simulink model "TorqueSteerCompensator"  (R2025b)
settings: Solver=VariableStepAuto  StartTime=0.0  StopTime=10.0  RelTol=1e-3
values from neighbouring files (symbols this model uses):
  Ke = 0.8    [TorqueSteerCompensator.mat]
  Kfb = 0.5    [TorqueSteerCompensator.mat]
  Kff = 1    [TorqueSteerCompensator.mat]
settings Model: Creator=sharm  LastModifiedBy=sharm

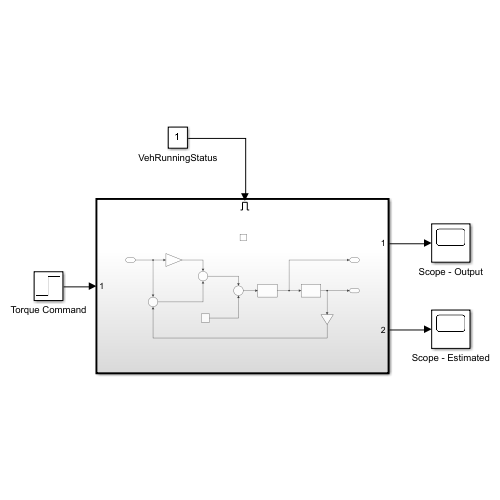
[thumbnail: Simulink's stored preview of the top-level diagram]
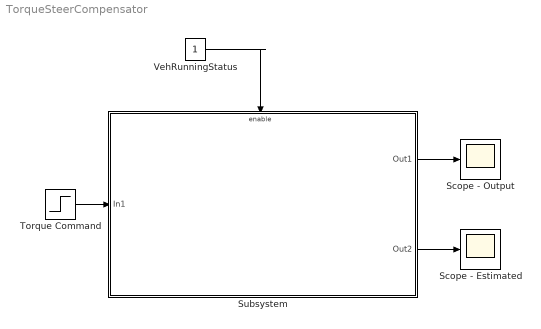
== system TorqueSteerCompensator ==
  Scope - Estimated : Scope
      settings: ActiveDisplayYMinimum=-0.16435887299849231  ActiveDisplayYMaximum=1.4792298569864311
  Scope - Output : Scope
      settings: ActiveDisplayYMinimum=-0.3828039560539751  ActiveDisplayYMaximum=1.9112315071928312
  Subsystem : Subsystem
  Torque Command : Step  SampleTime=0
  VehRunningStatus : Constant
  wires:
  Torque Command/1 -> Subsystem/1(In1)
  Subsystem/1(Out1) -> Scope - Output/1
  Subsystem/2(Out2) -> Scope - Estimated/1
  VehRunningStatus/1 -> Subsystem/Enable

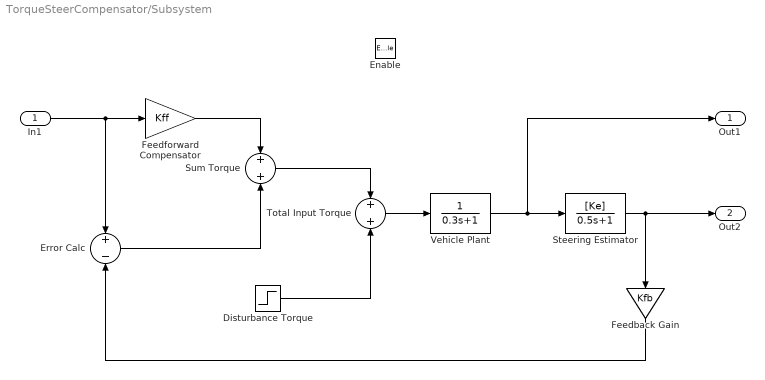
== system TorqueSteerCompensator/Subsystem ==
  In1 : Inport
  Enable : EnablePort
  Disturbance Torque : Step  Time=3  After=0.3  SampleTime=0
  Error Calc : Sum  Inputs=+-
  Feedback Gain : Gain  Gain=Kfb
  Feedforward Compensator : Gain  Gain=Kff
  Steering Estimator : TransferFcn  Numerator=[Ke]  Denominator=[0.5 1]
  Sum Torque : Sum
  Total Input Torque : Sum
  Vehicle Plant : TransferFcn  Denominator=[0.3 1]
  Out1 : Outport
  Out2 : Outport  Port=2
  wires:
  Disturbance Torque/1 -> Total Input Torque/2
  In1/1 -> Error Calc/1, Feedforward Compensator/1
  Sum Torque/1 -> Total Input Torque/1
  Error Calc/1 -> Sum Torque/2
  Steering Estimator/1 -> Out2/1, Feedback Gain/1
  Feedforward Compensator/1 -> Sum Torque/1
  Vehicle Plant/1 -> Out1/1, Steering Estimator/1
  Feedback Gain/1 -> Error Calc/2
  Total Input Torque/1 -> Vehicle Plant/1
